simulink model "grid_afe_n"  (R2026a)
settings: Solver=ode23tb  StopTime=simlength  FixedStep=tc  MaxStep=glb_time.tc
values from neighbouring files (symbols this model uses):
  afe_ctrl = ctrl_afe_setup(glb_time.ts_afe, grid_emu.omega_grid_nom)    [init_model.m]
  afe_pwm_phase_shift_mod1 = 0    [init_model.m]
  afe_pwm_phase_shift_mod2 = 0    [init_model.m]
  afe_pwm_phase_shift_mod3 = 0    [init_model.m]
  afe_pwm_phase_shift_mod4 = 0    [init_model.m]
  filters = setup_global_filters(glb_time.ts_afe, glb_time.ts_inv, glb_time.ts_dab, glb_time.tc)    [init_model.m]
  frt_data = frt_settings(test_index, test_subindex, asymmetric_error_type,      enable_frt_1, enable_frt_2, start_time_LVRT, deepPOSxi, deepPOSeta, deepNEGxi, deepNEGeta)    [init_model.m]
  glb_time = timing_setup(fpwm_afe, trgo_afe, fpwm_inv, trgo_inv, fpwm_single_phase_inv, trgo_single_phase_inv, fpwm_dab, trgo_dab,      fpwm_psfbc, trgo_psfbc, fpwm_isop_rail, trgo_isop_rail, fpwm_cllc, trgo_cllc, t_measure, tc_factor, tc_decimation, delay_pwm, dead_time_afe,      dead_time_inv, dead_time_single_phase_inv, dead_time_dab, dead_time_psfbc, dead_time_isop_rail, dead_time_cllc)    [init_model.m]
  grid_emu = grid_three_phase_emulator('Dyn11', delta_star, grid_nominal_power, application_voltage, us1, us2, fgrid,                  eq_grid_inductance, eq_grid_resistance, eta, ucc, i1m, p_iron, n1, n2, core_area, core_length, mur,                  up_xi_pu_ref, up_eta_pu_ref, un_xi_pu_ref, un_eta_pu_ref)    [init_model.m]
  i_react_pos_ref_2 = -ixi_ref_mod1*tan(acos(0.95))    [init_model.m]
  i_react_pos_ref_3 = ixi_ref_mod1*tan(acos(0.95))    [init_model.m]
  ixi_ref_mod1 = -0.85    [init_model.m]
  ixi_ref_mod2 = -0.85    [init_model.m]
  ixi_ref_mod3 = -0.85    [init_model.m]
  ixi_ref_mod4 = -0.85    [init_model.m]
  ki_align = 18    [init_model.m]
  kp_align = 0.25    [init_model.m]
  lim_down_align = -0.05    [init_model.m]
  lim_up_align = 0.05    [init_model.m]
  mavarage_filter_frequency_base_order = 2    [init_model.m]
  time_gain_afe_module_1 = 1.0002    [init_model.m]
  time_gain_afe_module_2 = 1.0015    [init_model.m]
  time_gain_afe_module_3 = 0.9988    [init_model.m]
  time_gain_afe_module_4 = 1.0020    (= 1.002)    [init_model.m]
  time_i_react_pos_ref_1 = start_time_LVRT + error_length + 0.335    [init_model.m]
  time_i_react_pos_ref_2 = time_i_react_pos_ref_1 + 0.5    (= 0.5)    [init_model.m]
  u_cm_comp_mod1 = 0    [init_model.m]
  u_cm_comp_mod2 = -1    [init_model.m]
  u_cm_comp_mod3 = -1    [init_model.m]
  u_cm_comp_mod4 = -1    [init_model.m]
undefined symbols (not defined in the file or in its folder): hwdata, magnitude
libraries: fl_lib x113, nesl_utility x75, moving_average_filter x40, moving_average_filter_cc x32, sl_discontinuities x12, linear_double_integrator_observer_ccaller x8, discrete_time_low_pass_filter x4, threephase_inductor_lib x4, dclink_for_two_levels x4, three_phase_pwm_modulator x4, three_phase_inverter_ideal_switch_based_model x4, three_phase_inverter_igbt_advanced_thermal_model x4
(part 8 of 19)

== system grid_afe_n/afe_abc_mod2/AFE_control/afe_control/current_ctrl/inner_current_ctrl ==
  In1 : Inport
  is_abc : Inport  Port=2
  Mux : Mux  Inputs=3
  Selector : Selector  InputPortWidth=3  IndexOptions=Index vector (dialog)  Indices=[1]  OutputSizes=1
  Selector1 : Selector  InputPortWidth=3  IndexOptions=Index vector (dialog)  Indices=[1]  OutputSizes=1
  Selector2 : Selector  InputPortWidth=3  IndexOptions=Index vector (dialog)  Indices=[2]  OutputSizes=1
  Selector3 : Selector  InputPortWidth=3  IndexOptions=Index vector (dialog)  Indices=[2]  OutputSizes=1
  Selector4 : Selector  InputPortWidth=3  IndexOptions=Index vector (dialog)  Indices=[3]  OutputSizes=1
  Selector5 : Selector  InputPortWidth=3  IndexOptions=Index vector (dialog)  Indices=[3]  OutputSizes=1
  isa_ref/isa : Scope  NumInputPorts=2
      settings: ActiveDisplayYMinimum=-3.12274169921875  ActiveDisplayYMaximum=3.67108154296875
  isb_ref/isb : Scope  NumInputPorts=2
      settings: ActiveDisplayYMinimum=-2.378662109375  ActiveDisplayYMaximum=2.814208984375  DataLoggingVariableName=ScopeData2
  isc_ref/isc : Scope  NumInputPorts=2
      settings: ActiveDisplayYMinimum=-2.90966796875  ActiveDisplayYMaximum=2.88134765625  DataLoggingVariableName=ScopeData3
  rpi_phase_a : Subsystem
  rpi_phase_b : Subsystem
  rpi_phase_c : Subsystem
  zero_current_ctrl : Subsystem
  uabg : Outport  VectorParamsAs1DForOutWhenUnconnected=off
  tag scope: isa=scoped, isa_ref=scoped, isb=scoped, isb_ref=scoped, isc=scoped, isc_ref=scoped
  wires:
  zero_current_ctrl/1(u_ctrl_out) -> uabg/1
  Mux/1 -> zero_current_ctrl/1(d_abc)  "d_abc"
  rpi_phase_c/1(Out1) -> Mux/3  "dc"
  rpi_phase_b/1(Out1) -> Mux/2  "db"
  rpi_phase_a/1(Out1) -> Mux/1  "da"
  Selector5/1 -> isc_ref/isc/2, [isc], rpi_phase_c/2(In2)  "isc"
  Selector4/1 -> isc_ref/isc/1, [isc_ref], rpi_phase_c/1(In1)  "isc_ref"
  Selector3/1 -> isb_ref/isb/2, [isb], rpi_phase_b/2(In2)  "isb"
  Selector2/1 -> isb_ref/isb/1, [isb_ref], rpi_phase_b/1(In1)  "isb_ref"
  Selector1/1 -> rpi_phase_a/2(In2), isa_ref/isa/2, [isa]  "isa"
  Selector/1 -> rpi_phase_a/1(In1), isa_ref/isa/1, [isa_ref]  "isa_ref"
  is_abc/1 -> Selector1/1, Selector3/1, Selector5/1  "id_abc"
  In1/1 -> Selector/1, Selector2/1, Selector4/1  "id_abc_ref"

== system grid_afe_n/afe_abc_mod2/AFE_control/afe_control/current_ctrl/xieta2abc ==
  pos_xi : Inport
  pos_eta : Inport  Port=2
  neg_xi : Inport  Port=3
  neg_eta : Inport  Port=4
  phase : Inport  Port=5
  MATLAB Function2 : MATLAB Function  TreatAsAtomicUnit=on
  Mux : Mux  Inputs=3
  Negative Sequence : MATLAB Function  TreatAsAtomicUnit=on
  Positive Sequence : MATLAB Function  TreatAsAtomicUnit=on
  Sum : Sum  Inputs=|++
  Sum1 : Sum  Inputs=|++
  i_abc : Outport
  wires:
  Mux/1 -> i_abc/1  "i_abc"
  pos_eta/1 -> Positive Sequence/2(eta)
  pos_xi/1 -> Positive Sequence/1(xi)
  neg_xi/1 -> Negative Sequence/1(xi)
  Sum1/1 -> MATLAB Function2/2(beta)
  MATLAB Function2/2(b) -> Mux/2  "i_b"
  Negative Sequence/2(beta) -> Sum1/2
  Positive Sequence/1(alpha) -> Sum/1
  Negative Sequence/1(alpha) -> Sum/2
  MATLAB Function2/3(c) -> Mux/3  "i_c"
  phase/1 -> Positive Sequence/3(phase), Negative Sequence/3(phase)
  Sum/1 -> MATLAB Function2/1(alpha)
  Positive Sequence/2(beta) -> Sum1/1
  MATLAB Function2/1(a) -> Mux/1  "i_a"
  neg_eta/1 -> Negative Sequence/2(eta)

== system grid_afe_n/afe_abc_mod2/AFE_control/afe_control/data_to_worspace_module_1/dq_pll ==
  Bus Creator1 : BusCreator  Inputs=8
  dqPLLs : Outport
  wires:
  [phase_grid_fht_simulink_pll] -> Bus Creator1/5  "phase_grid_fht_simulink_pll"
  [omega_grid_fht_simulink_pll] -> Bus Creator1/6  "omega_grid_fht_simulink_pll"
  [omega_grid_fhtsr_dqpll] -> Bus Creator1/8  "omega_grid_fhtsr_dqpll"
  [phase_grid_fhtsr_dqpll] -> Bus Creator1/7  "phase_grid_fhtsr_dqpll"
  [omega_grid_dqpll_ccaller] -> Bus Creator1/4  "omega_grid_dqpll_ccaller"
  [phase_grid_dqpll_ccaller] -> Bus Creator1/3  "phase_grid_dqpll_ccaller"
  [omega_grid_pll_pu] -> Bus Creator1/2  "omega_grid_pu_dqpll"
  [phase_grid_pll] -> Bus Creator1/1  "phase_grid_dqpll"
  Bus Creator1/1 -> dqPLLs/1

== system grid_afe_n/afe_abc_mod2/AFE_control/afe_control/data_to_worspace_module_1/inner_current_tracking ==
  Bus Creator1 : BusCreator  Inputs=11
  m_inner_current_tracking : Outport
  wires:
  Bus Creator1/1 -> m_inner_current_tracking/1
  [isc_ref] -> Bus Creator1/7  "isc_pu_ref"
  [iz_ctrl_out] -> Bus Creator1/11  "iz_ctrl_out"
  [isb_ref] -> Bus Creator1/5  "isb_pu_ref"
  [isb] -> Bus Creator1/6  "isb_pu"
  [iz_pu_ref] -> Bus Creator1/9  "iz_pu_ref"
  [id_xi_pu] -> Bus Creator1/1  "i_xi_pu"
  [isa] -> Bus Creator1/4  "isa_pu"
  [isa_ref] -> Bus Creator1/3  "isa_pu_ref"
  [isc] -> Bus Creator1/8  "isc_pu"
  [id_eta_pu] -> Bus Creator1/2  "i_eta_pu"
  [iz_pu] -> Bus Creator1/10  "iz_pu"

== system grid_afe_n/afe_abc_mod2/AFE_control/afe_control/data_to_worspace_module_1/pwr_meter ==
  Bus Creator1 : BusCreator  Inputs=4
  m_pwr_meter : Outport
  wires:
  [i_grid_pu_rms] -> Bus Creator1/1  "i_grid_pu_rms"
  [pwr_react_grid] -> Bus Creator1/4  "pwr_react_grid"
  [pwr_act_grid] -> Bus Creator1/3  "pwr_act_grid"
  Bus Creator1/1 -> m_pwr_meter/1
  [u_grid_pu_rms] -> Bus Creator1/2  "u_grid_pu_rms"

== system grid_afe_n/afe_abc_mod2/AFE_control/afe_control/data_to_worspace_module_1/sequences_data ==
  Bus Creator1 : BusCreator  Inputs=11
  Bus Selector : BusSelector  OutputSignals=i_grid_pos_eta_ref,i_grid_neg_eta_ref,i_grid_neg_xi_ref
  m_seq : Outport
  wires:
  Bus Creator1/1 -> m_seq/1
  [i_grid_seq_ref] -> Bus Selector/1
  Bus Selector/3 -> Bus Creator1/3  "<i_grid_neg_xi_ref>"
  Bus Selector/2 -> Bus Creator1/2  "<i_grid_neg_eta_ref>"
  Bus Selector/1 -> Bus Creator1/1  "<i_grid_pos_eta_ref>"
  [v_grid_pos_xi_avg] -> Bus Creator1/4  "v_grid_pos_xi_avg"
  [v_grid_pos_eta_avg] -> Bus Creator1/5  "v_grid_pos_eta_avg"
  [v_grid_neg_xi_avg] -> Bus Creator1/6  "v_grid_neg_xi_avg"
  [v_grid_neg_eta_avg] -> Bus Creator1/7  "v_grid_neg_eta_avg"
  [i_grid_pos_xi_avg] -> Bus Creator1/8  "i_grid_pos_xi_avg"
  [i_grid_pos_eta_avg] -> Bus Creator1/9  "i_grid_pos_eta_avg"
  [i_grid_neg_xi_avg] -> Bus Creator1/10  "i_grid_neg_xi_avg"
  [i_grid_neg_eta_avg] -> Bus Creator1/11  "i_grid_neg_eta_avg"

== system grid_afe_n/afe_abc_mod2/AFE_control/afe_control/grid_current_sequences_and_reactive_pwr_ctrl/current_sequence_avg ==
  i_grid_pos_xi : Inport
  i_grid_pos_eta : Inport  Port=2
  i_grid_neg_xi : Inport  Port=3
  i_grid_neg_eta : Inport  Port=4
  Variant Source{,1..3} (4 alike) : VariantSource  VariantControls={use_moving_average_from_ccaller_mod3 == 1, use_moving_average_from_ccaller_mod3 == 0}
  average_filter : Subsystem
  average_filter_ccaller : Subsystem
  i_grid_pos_xi_avg : Outport
  i_grid_pos_eta_avg : Outport  Port=2
  i_grid_neg_xi_avg : Outport  Port=3
  i_grid_neg_eta_avg : Outport  Port=4
  wires:
  average_filter_ccaller/4(i_grid_neg_eta_avg) -> Variant Source3/1
  average_filter_ccaller/3(i_grid_neg_xi_avg) -> Variant Source2/1
  average_filter_ccaller/2(i_grid_pos_eta_avg) -> Variant Source1/1
  average_filter/4(i_grid_neg_eta_avg) -> Variant Source3/2
  average_filter/3(i_grid_neg_xi_avg) -> Variant Source2/2
  average_filter/2(i_grid_pos_eta_avg) -> Variant Source1/2
  average_filter/1(i_grid_pos_xi_avg) -> Variant Source/2
  average_filter_ccaller/1(i_grid_pos_xi_avg) -> Variant Source/1
  Variant Source1/1 -> i_grid_pos_eta_avg/1
  Variant Source2/1 -> i_grid_neg_xi_avg/1
  Variant Source3/1 -> i_grid_neg_eta_avg/1
  Variant Source/1 -> i_grid_pos_xi_avg/1
  i_grid_neg_eta/1 -> average_filter_ccaller/4(i_grid_neg_eta), average_filter/4(i_grid_neg_eta)
  i_grid_neg_xi/1 -> average_filter_ccaller/3(i_grid_neg_xi), average_filter/3(i_grid_neg_xi)
  i_grid_pos_eta/1 -> average_filter_ccaller/2(i_grid_pos_eta), average_filter/2(i_grid_pos_eta)
  i_grid_pos_xi/1 -> average_filter_ccaller/1(i_grid_pos_xi), average_filter/1(i_grid_pos_xi)

== system grid_afe_n/afe_abc_mod2/AFE_control/afe_control/grid_current_sequences_and_reactive_pwr_ctrl/grid_current_sampling_and_alpha_beta_transformation ==
  ig_abc : Inport
  i_abc2alphabeta : MATLAB Function  TreatAsAtomicUnit=on
  i_grid_alpha : Outport
  i_grid_beta : Outport  Port=2
  wires:
  ig_abc/1 -> i_abc2alphabeta/1(i_abc)
  i_abc2alphabeta/1(alpha) -> i_grid_alpha/1  "i_grid_alpha"
  i_abc2alphabeta/2(beta) -> i_grid_beta/1  "i_grid_beta"

== system grid_afe_n/afe_abc_mod2/AFE_control/afe_control/grid_current_sequences_and_reactive_pwr_ctrl/i_alphabeta2xieta ==
  alpha : Inport
  beta : Inport  Port=2
  gamma : Inport  Port=3
  MATLAB Function : MATLAB Function  TreatAsAtomicUnit=on
  MATLAB Function1 : MATLAB Function  TreatAsAtomicUnit=on
  xi : Outport
  v_grid_pos_eta : Outport  Port=2
  v_grid_neg_xi : Outport  Port=3
  e : Outport  Port=4
  wires:
  MATLAB Function/1(xi) -> xi/1  "i_grid_pos_xi"
  MATLAB Function1/2(eta) -> e/1  "i_grid_neg_eta"
  MATLAB Function1/1(xi) -> v_grid_neg_xi/1  "i_grid_neg_xi"
  MATLAB Function/2(eta) -> v_grid_pos_eta/1  "i_grid_pos_eta"
  gamma/1 -> MATLAB Function/3(gamma), MATLAB Function1/3(gamma)  "gamma_grid"
  beta/1 -> MATLAB Function/2(beta), MATLAB Function1/2(beta)  "i_grid_beta"
  alpha/1 -> MATLAB Function/1(alpha), MATLAB Function1/1(alpha)  "i_grid_alpha"

== system grid_afe_n/afe_abc_mod2/AFE_control/afe_control/grid_current_sequences_and_reactive_pwr_ctrl/sequences_current_control ==
  i_pos_xi : Inport
  i_pos_eta : Inport  Port=2
  i_neg_xi : Inport  Port=3
  i_neg_eta : Inport  Port=4
  Bus Selector : BusSelector  OutputSignals=i_grid_pos_eta_ref,i_grid_neg_eta_ref,i_grid_neg_xi_ref
  Constant : Constant  Value=0
  Constant1 : Constant  Value=0
  Constant2 : Constant  Value=0
  Gain : Gain  Gain=-1
  Gain1 : Gain  Gain=-1
  Gain2 : Gain  Gain=-1
  Negative-Seq. eta-Control : Subsystem
  Negative-Seq. xi-Control : Subsystem
  Positive-Seq. eta-Control : Subsystem
  Sum : Sum  Inputs=|+-
  Sum1 : Sum  Inputs=|+-
  Sum2 : Sum  Inputs=|+-
  Terminator : Terminator
  i_neg_eta_ref/i_neg_eta : Scope  NumInputPorts=2
      settings: ActiveDisplayYMinimum=-1  ActiveDisplayYMaximum=1  DataLoggingVariableName=ScopeData6
  i_neg_xi_ref/i_neg_xi : Scope  NumInputPorts=2
      settings: ActiveDisplayYMinimum=-2.0072433506888805  ActiveDisplayYMaximum=0.71326150187789183  DataLoggingVariableName=ScopeData7
  i_pos_eta_ref/i_pos_eta : Scope  NumInputPorts=2
      settings: ActiveDisplayYMinimum=-2.9962328913117955  ActiveDisplayYMaximum=0.9969886390149818  DataLoggingVariableName=ScopeData5
  tag scope: i_stack_neg_eta_ref=scoped, i_stack_neg_xi_ref=scoped, i_stack_pos_eta_ref=scoped
  wires:
  Negative-Seq. xi-Control/1(u) -> [i_stack_neg_xi_ref]
  Negative-Seq. eta-Control/1(u) -> [i_stack_neg_eta_ref]
  Positive-Seq. eta-Control/1(u) -> [i_stack_pos_eta_ref]
  Gain2/1 -> Negative-Seq. xi-Control/2(e)
  Gain1/1 -> Negative-Seq. eta-Control/2(e)
  Gain/1 -> Positive-Seq. eta-Control/2(e)
  i_neg_xi/1 -> Sum2/2, i_neg_xi_ref/i_neg_xi/2  "i_neg_xi"
  i_neg_eta/1 -> i_neg_eta_ref/i_neg_eta/2, Sum1/2  "i_neg_eta"
  i_pos_eta/1 -> Sum/2, i_pos_eta_ref/i_pos_eta/2  "i_pos_eta"
  Sum/1 -> Gain/1
  Sum1/1 -> Gain1/1
  Sum2/1 -> Gain2/1
  Bus Selector/3 -> Sum2/1, i_neg_xi_ref/i_neg_xi/1  "<i_grid_neg_xi_ref>"
  Bus Selector/2 -> Sum1/1, i_neg_eta_ref/i_neg_eta/1  "<i_grid_neg_eta_ref>"
  Bus Selector/1 -> Sum/1, i_pos_eta_ref/i_pos_eta/1  "<i_grid_pos_eta_ref>"
  [i_grid_seq_ref] -> Bus Selector/1
  i_pos_xi/1 -> Terminator/1
  Constant/1 -> Positive-Seq. eta-Control/1(ff)
  Constant1/1 -> Negative-Seq. eta-Control/1(ff)
  Constant2/1 -> Negative-Seq. xi-Control/1(ff)

== system grid_afe_n/afe_abc_mod2/AFE_control/afe_control/grid_voltage_phase_lock_loops/FHT-PLL ==
  ug_abc_pu : Inport
  pll_stageA : Subsystem
  pll_stageB : Subsystem
  gamma_grid_fht_pll : Outport
  omega_grid_fht_pll : Outport  Port=2
  wires:
  pll_stageB/1(gamma_grid_ddsrf_pll) -> pll_stageA/1(gamma_grid), gamma_grid_fht_pll/1
  pll_stageA/2(u_grid_eta) -> pll_stageB/2(u_grid_pos_eta)  "u_grid_pos_eta"
  pll_stageA/1(u_grid_xi) -> pll_stageB/1(u_grid_pos_xi)  "u_grid_pos_xi"
  pll_stageB/2(omega_grid_ddsrf_pll) -> omega_grid_fht_pll/1
  ug_abc_pu/1 -> pll_stageA/2(ug_abc_pu)

== system grid_afe_n/afe_abc_mod2/AFE_control/afe_control/grid_voltage_phase_lock_loops/FHT-PLL_simulink ==
  ug_abc_pu : Inport
  Goto Tag Visibility55 : GotoTagVisibility  GotoTag=Vgrid_unorm_fht_simulink
  pll_stageA : Subsystem
  pll_stageB : Subsystem
  gamma_grid_fht_pll : Outport
  omega_grid_fht_pll : Outport  Port=2
  wires:
  pll_stageB/1(gamma_grid_ddsrf_pll) -> pll_stageA/1(gamma_grid), gamma_grid_fht_pll/1
  pll_stageA/2(u_grid_eta) -> pll_stageB/2(u_grid_pos_eta)  "u_grid_pos_eta"
  pll_stageA/1(u_grid_xi) -> pll_stageB/1(u_grid_pos_xi)  "u_grid_pos_xi"
  pll_stageB/2(omega_grid_ddsrf_pll) -> omega_grid_fht_pll/1
  ug_abc_pu/1 -> pll_stageA/2(ug_abc_pu)

== system grid_afe_n/afe_abc_mod2/AFE_control/afe_control/grid_voltage_phase_lock_loops/dq_pll ==
  ug_abc_pu : Inport
  Goto Tag Visibility1 : GotoTagVisibility  GotoTag=Vgrid_unorm_dqpll
  pll_stageA : Subsystem
  pll_stageB : Subsystem
  phase_grid_dqpll : Outport
  omega_grid_pu_dqpll : Outport  Port=2
  wires:
  ug_abc_pu/1 -> pll_stageA/2(ug_abc)
  pll_stageB/2(omega_grid_pu_pll) -> omega_grid_pu_dqpll/1
  pll_stageA/1(u_grid_pos_xi) -> pll_stageB/1(u_grid_pos_xi)  "u_grid_pos_xi"
  pll_stageB/1(phase_grid_pll) -> pll_stageA/1(phase_grid), phase_grid_dqpll/1
  pll_stageA/2(u_grid_pos_eta) -> pll_stageB/2(u_grid_pos_eta)  "u_grid_pos_eta"

== system grid_afe_n/afe_abc_mod2/AFE_control/afe_control/grid_voltage_phase_lock_loops/dq_pll_ccaller ==
  ug_abc_pu : Inport
  Bus Selector : BusSelector  OutputSignals=omega_pu_hat,gamma_hat,u_grid_xi,u_grid_eta,dqpll_pll_state
  C Caller : CCaller  FunctionName=dqpll_grid_process_simulink  PortSpecificationStruct="%)30     .    N H   8    (     @         %    \"     8    !     0         %  0 \"0    $    _    07)G3F%M90  4&]R=$YA;64 4V-O<&4     26YD97@     5'EP90      4VEZ90      27-';&]B86P   X    P    !@    @    $          4    (     0    ,    !         !   P!O=70 #@   #     &    \"     0         !0    @    !     P    $         $  # &]U=  .    .     8    (    !          %    \"     $    &     0         0   ...(+3319 chars)"
  Constant : Constant  Value=glb_time.ts_afe
  Data Type Conversion{1..2,4..5} (4 alike) : DataTypeConversion  OutDataTypeStr=single  SaturateOnIntegerOverflow=off  RndMeth=Floor
  Data Type Conversion{6..10} (5 alike) : DataTypeConversion  OutDataTypeStr=double  SaturateOnIntegerOverflow=off  RndMeth=Floor
  Data Type Conversion3 : DataTypeConversion  OutDataTypeStr=uint8  SaturateOnIntegerOverflow=off  RndMeth=Floor
  Demux : Demux  Outputs=3
  Step : Step  Time=0.01  InitialValue=1  FinalValue=0
  first_harmonic_tracker : Scope  NumInputPorts=3
      settings: ActiveDisplayYMinimum=-1.7184470891952515  ActiveDisplayYMaximum=1.8384636640548706
  first_harmonic_tracker_phase_u : Subsystem
  first_harmonic_tracker_phase_v : Subsystem
  first_harmonic_tracker_phase_w : Subsystem
  gamma_hat : Outport  VectorParamsAs1DForOutWhenUnconnected=off
  omega_pu_hat : Outport  Port=2  VectorParamsAs1DForOutWhenUnconnected=off
  dqpll_uxi : Outport  Port=3  VectorParamsAs1DForOutWhenUnconnected=off
  dqpll_ueta : Outport  Port=4  VectorParamsAs1DForOutWhenUnconnected=off
  dqpll_state : Outport  Port=5  VectorParamsAs1DForOutWhenUnconnected=off
  wires:
  first_harmonic_tracker_phase_w/1(u_hat) -> Data Type Conversion5/1, first_harmonic_tracker/3  "tracker_phase_w"
  first_harmonic_tracker_phase_v/1(u_hat) -> Data Type Conversion4/1, first_harmonic_tracker/2  "tracker_phase_v"
  first_harmonic_tracker_phase_u/1(u_hat) -> Data Type Conversion2/1, first_harmonic_tracker/1  "tracker_phase_u"
  Data Type Conversion6/1 -> omega_pu_hat/1
  Demux/3 -> first_harmonic_tracker_phase_w/1(u)
  Demux/2 -> first_harmonic_tracker_phase_v/1(u)
  Demux/1 -> first_harmonic_tracker_phase_u/1(u)
  ug_abc_pu/1 -> Demux/1
  Data Type Conversion9/1 -> dqpll_ueta/1
  Data Type Conversion8/1 -> dqpll_uxi/1
  Data Type Conversion10/1 -> dqpll_state/1
  Data Type Conversion7/1 -> gamma_hat/1
  Bus Selector/5 -> Data Type Conversion10/1  "<dqpll_pll_state>"
  Bus Selector/4 -> Data Type Conversion9/1  "<u_grid_eta>"
  Bus Selector/3 -> Data Type Conversion8/1  "<u_grid_xi>"
  Bus Selector/2 -> Data Type Conversion7/1  "<gamma_hat>"
  Bus Selector/1 -> Data Type Conversion6/1  "<omega_pu_hat>"
  C Caller/1 -> Bus Selector/1
  Data Type Conversion1/1 -> C Caller/5
  Data Type Conversion5/1 -> C Caller/4
  Data Type Conversion4/1 -> C Caller/3
  Data Type Conversion2/1 -> C Caller/2
  Data Type Conversion3/1 -> C Caller/1
  Constant/1 -> Data Type Conversion1/1
  Step/1 -> Data Type Conversion3/1

== system grid_afe_n/afe_abc_mod2/AFE_control/afe_control/grid_voltage_sequences/grid_voltage_sampling_and_alpha_beta_transformation ==
  v_abc : Inport
  v_abc2alphabeta : MATLAB Function  TreatAsAtomicUnit=on
  u_grid_alpha : Outport
  u_grid_beta : Outport  Port=2
  wires:
  v_abc/1 -> v_abc2alphabeta/1(v_abc)
  v_abc2alphabeta/2(beta) -> u_grid_beta/1  "u_grid_beta"
  v_abc2alphabeta/1(alpha) -> u_grid_alpha/1  "u_grid_alpha"

== system grid_afe_n/afe_abc_mod2/AFE_control/afe_control/grid_voltage_sequences/v_alphabeta2xieta ==
  alpha : Inport
  beta : Inport  Port=2
  gamma : Inport  Port=3
  MATLAB Function : MATLAB Function  TreatAsAtomicUnit=on
  MATLAB Function1 : MATLAB Function  TreatAsAtomicUnit=on
  xi : Outport
  eta : Outport  Port=2
  v_grid_neg_xi : Outport  Port=3
  v_grid_neg_eta : Outport  Port=4
  wires:
  MATLAB Function1/2(eta) -> v_grid_neg_eta/1  "u_grid_neg_eta"
  MATLAB Function1/1(xi) -> v_grid_neg_xi/1  "u_grid_neg_xi"
  MATLAB Function/2(eta) -> eta/1  "u_grid_pos_eta"
  MATLAB Function/1(xi) -> xi/1  "u_grid_pos_xi"
  gamma/1 -> MATLAB Function/3(gamma), MATLAB Function1/3(gamma)  "gamma_grid"
  beta/1 -> MATLAB Function/2(beta), MATLAB Function1/2(beta)  "u_grid_beta"
  alpha/1 -> MATLAB Function/1(alpha), MATLAB Function1/1(alpha)  "u_grid_alpha"

== system grid_afe_n/afe_abc_mod2/AFE_control/afe_control/grid_voltage_sequences/voltage_sequence_avg ==
  v_grid_pos_xi : Inport
  v_grid_pos_eta : Inport  Port=2
  v_grid_neg_xi : Inport  Port=3
  v_grid_neg_eta : Inport  Port=4
  Variant Source{1..4} (4 alike) : VariantSource  VariantControls={use_moving_average_from_ccaller_mod2 == 1, use_moving_average_from_ccaller_mod2 == 0}
  average_filter : Subsystem
  average_filter_ccaller : Subsystem
  v_grid_pos_xi_avg : Outport
  v_grid_pos_eta_avg : Outport  Port=2
  v_grid_neg_xi_avg : Outport  Port=3
  v_grid_neg_eta_avg : Outport  Port=4
  wires:
  average_filter/4(v_grid_neg_eta_avg) -> Variant Source3/2
  average_filter/3(v_grid_neg_xi_avg) -> Variant Source2/2
  average_filter/2(v_grid_pos_eta_avg) -> Variant Source1/2
  average_filter/1(v_grid_pos_xi_avg) -> Variant Source4/2
  average_filter_ccaller/4(v_grid_neg_eta_avg) -> Variant Source3/1
  average_filter_ccaller/3(v_grid_neg_xi_avg) -> Variant Source2/1
  average_filter_ccaller/2(v_grid_pos_eta_avg) -> Variant Source1/1
  average_filter_ccaller/1(v_grid_pos_xi_avg) -> Variant Source4/1
  Variant Source3/1 -> v_grid_neg_eta_avg/1
  Variant Source2/1 -> v_grid_neg_xi_avg/1
  Variant Source1/1 -> v_grid_pos_eta_avg/1
  Variant Source4/1 -> v_grid_pos_xi_avg/1
  v_grid_neg_eta/1 -> average_filter/4(v_grid_neg_eta), average_filter_ccaller/4(v_grid_neg_eta)
  v_grid_neg_xi/1 -> average_filter/3(v_grid_neg_xi), average_filter_ccaller/3(v_grid_neg_xi)
  v_grid_pos_eta/1 -> average_filter/2(v_grid_pos_eta), average_filter_ccaller/2(v_grid_pos_eta)
  v_grid_pos_xi/1 -> average_filter_ccaller/1(v_grid_pos_xi), average_filter/1(v_grid_pos_xi)

== system grid_afe_n/afe_abc_mod2/AFE_control/afe_control/ig afe quantizzation and one step delay/ig afe quantizzation and one step delay ==
  ig_u_pu : Inport
  ig_v_pu : Inport  Port=2
  ig_w_pu : Inport  Port=3
  Gain4 : Gain  Gain=-1
  Gain5 : Gain  Gain=-1
  Gain6 : Gain  Gain=-1
  Quantizer1 : Quantizer  QuantizationInterval=adc_quantization
  Quantizer2 : Quantizer  QuantizationInterval=adc_quantization
  Quantizer4 : Quantizer  QuantizationInterval=adc_quantization
  Unit Delay : UnitDelay  SampleTime=-1
  Unit Delay1 : UnitDelay  SampleTime=-1
  Unit Delay2 : UnitDelay  SampleTime=-1
  Zero-Order Hold : ZeroOrderHold  SampleTime=-1
  Zero-Order Hold1 : ZeroOrderHold  SampleTime=-1
  Zero-Order Hold2 : ZeroOrderHold  SampleTime=-1
  igd_u_pu : Outport
  igd_v_pu : Outport  Port=2
  igd_w_pu : Outport  Port=3
  wires:
  Zero-Order Hold2/1 -> Quantizer2/1
  Zero-Order Hold1/1 -> Quantizer1/1
  Zero-Order Hold/1 -> Quantizer4/1
  Gain6/1 -> igd_w_pu/1
  Gain5/1 -> igd_v_pu/1
  Gain4/1 -> igd_u_pu/1
  Unit Delay2/1 -> Gain6/1
  Unit Delay1/1 -> Gain5/1
  Unit Delay/1 -> Gain4/1
  ig_w_pu/1 -> Zero-Order Hold2/1
  ig_v_pu/1 -> Zero-Order Hold1/1
  ig_u_pu/1 -> Zero-Order Hold/1
  Quantizer2/1 -> Unit Delay2/1
  Quantizer4/1 -> Unit Delay/1
  Quantizer1/1 -> Unit Delay1/1

== system grid_afe_n/afe_abc_mod2/AFE_control/afe_control/instantaneus_power/abc2alphabeta ==
  a : Inport
  b : Inport  Port=2
  c : Inport  Port=3
  Gain1 : Gain  Gain=-1/2
  Gain11 : Gain  Gain=-1/2
  Gain2 : Gain  Gain=0
  Gain3 : Gain  Gain=sqrt(3)/2
  Gain4 : Gain  Gain=-sqrt(3)/2
  Gain8 : Gain  Gain=2/3
  Gain9 : Gain  Gain=2/3
  Sum : Sum  Inputs=+++
  Sum1 : Sum  Inputs=+++
  "alpha " : Outport  VectorParamsAs1DForOutWhenUnconnected=off
  "beta " : Outport  Port=2  VectorParamsAs1DForOutWhenUnconnected=off
  wires:
  a/1 -> Sum/1, Gain2/1
  Gain1/1 -> Sum/3
  b/1 -> Gain11/1, Gain3/1
  Gain9/1 -> "beta "/1
  c/1 -> Gain1/1, Gain4/1
  Sum/1 -> Gain8/1
  Gain8/1 -> "alpha "/1
  Sum1/1 -> Gain9/1
  Gain4/1 -> Sum1/3
  Gain11/1 -> Sum/2
  Gain2/1 -> Sum1/1
  Gain3/1 -> Sum1/2

== system grid_afe_n/afe_abc_mod2/AFE_control/afe_control/instantaneus_power/abc2alphabeta  ==
  a : Inport
  b : Inport  Port=2
  c : Inport  Port=3
  Gain1 : Gain  Gain=-1/2
  Gain11 : Gain  Gain=-1/2
  Gain2 : Gain  Gain=0
  Gain3 : Gain  Gain=sqrt(3)/2
  Gain4 : Gain  Gain=-sqrt(3)/2
  Gain8 : Gain  Gain=2/3
  Gain9 : Gain  Gain=2/3
  Sum : Sum  Inputs=+++
  Sum1 : Sum  Inputs=+++
  "alpha " : Outport  VectorParamsAs1DForOutWhenUnconnected=off
  "beta " : Outport  Port=2  VectorParamsAs1DForOutWhenUnconnected=off
  wires:
  b/1 -> Gain3/1, Gain11/1
  Gain8/1 -> "alpha "/1
  Gain4/1 -> Sum1/3
  Gain3/1 -> Sum1/2
  Gain1/1 -> Sum/3
  Sum1/1 -> Gain9/1
  Sum/1 -> Gain8/1
  c/1 -> Gain4/1, Gain1/1
  Gain11/1 -> Sum/2
  Gain9/1 -> "beta "/1
  Gain2/1 -> Sum1/1
  a/1 -> Gain2/1, Sum/1

== system grid_afe_n/afe_abc_mod2/AFE_control/afe_control/instantaneus_power/moving_avarage_p ==
  in : Inport
  Gain : Gain  Gain=afe_ctrl.rms.n1-1
  Gain1 : Gain  Gain=1/afe_ctrl.rms.n1
  Sum : Sum  Inputs=|++
  Unit Delay : UnitDelay  SampleTime=-1
  out : Outport  VectorParamsAs1DForOutWhenUnconnected=off
  wires:
  Sum/1 -> Gain1/1
  Unit Delay/1 -> Gain/1
  in/1 -> Sum/1
  Gain1/1 -> Unit Delay/1, out/1
  Gain/1 -> Sum/2

== system grid_afe_n/afe_abc_mod2/AFE_control/afe_control/instantaneus_power/moving_avarage_q ==
  in : Inport
  Gain : Gain  Gain=afe_ctrl.rms.n1-1
  Gain1 : Gain  Gain=1/afe_ctrl.rms.n1
  Sum : Sum  Inputs=|++
  Unit Delay : UnitDelay  SampleTime=-1
  out : Outport  VectorParamsAs1DForOutWhenUnconnected=off
  wires:
  Gain/1 -> Sum/2
  Gain1/1 -> out/1, Unit Delay/1
  in/1 -> Sum/1
  Unit Delay/1 -> Gain/1
  Sum/1 -> Gain1/1

== system grid_afe_n/afe_abc_mod2/AFE_control/afe_control/instantaneus_power/rms ==
  In1 : Inport
  Gain : Gain  Gain=afe_ctrl.rms.n10-1
  Gain1 : Gain  Gain=1/afe_ctrl.rms.n10
  Math Function : Math  Operator=magnitude^2  SignedPower=on
  Sqrt : Sqrt
  Sum : Sum  Inputs=|++
  Unit Delay : UnitDelay  SampleTime=-1
  Out1 : Outport  VectorParamsAs1DForOutWhenUnconnected=off
  wires:
  Gain/1 -> Sum/2
  Sqrt/1 -> Out1/1
  Math Function/1 -> Sum/1
  Unit Delay/1 -> Gain/1
  Gain1/1 -> Unit Delay/1, Sqrt/1
  Sum/1 -> Gain1/1
  In1/1 -> Math Function/1

== system grid_afe_n/afe_abc_mod2/AFE_control/afe_control/instantaneus_power/rms1 ==
  In1 : Inport
  Gain : Gain  Gain=afe_ctrl.rms.n10-1
  Gain1 : Gain  Gain=1/afe_ctrl.rms.n10
  Math Function : Math  Operator=magnitude^2  SignedPower=on
  Sqrt : Sqrt
  Sum : Sum  Inputs=|++
  Unit Delay : UnitDelay  SampleTime=-1
  Out1 : Outport  VectorParamsAs1DForOutWhenUnconnected=off
  wires:
  In1/1 -> Math Function/1
  Sum/1 -> Gain1/1
  Gain1/1 -> Sqrt/1, Unit Delay/1
  Unit Delay/1 -> Gain/1
  Math Function/1 -> Sum/1
  Sqrt/1 -> Out1/1
  Gain/1 -> Sum/2

== system grid_afe_n/afe_abc_mod2/AFE_control/afe_control/instantaneus_power/rms2 ==
  In1 : Inport
  Gain : Gain  Gain=afe_ctrl.rms.n10-1
  Gain1 : Gain  Gain=1/afe_ctrl.rms.n10
  Math Function : Math  Operator=magnitude^2  SignedPower=on
  Sqrt : Sqrt
  Sum : Sum  Inputs=|++
  Unit Delay : UnitDelay  SampleTime=-1
  Out1 : Outport  VectorParamsAs1DForOutWhenUnconnected=off
  wires:
  Gain/1 -> Sum/2
  Sqrt/1 -> Out1/1
  Math Function/1 -> Sum/1
  Unit Delay/1 -> Gain/1
  Gain1/1 -> Unit Delay/1, Sqrt/1
  Sum/1 -> Gain1/1
  In1/1 -> Math Function/1

== system grid_afe_n/afe_abc_mod2/AFE_control/afe_control/instantaneus_power/rms3 ==
  In1 : Inport
  Gain : Gain  Gain=afe_ctrl.rms.n10-1
  Gain1 : Gain  Gain=1/afe_ctrl.rms.n10
  Math Function : Math  Operator=magnitude^2  SignedPower=on
  Sqrt : Sqrt
  Sum : Sum  Inputs=|++
  Unit Delay : UnitDelay  SampleTime=-1
  Out1 : Outport  VectorParamsAs1DForOutWhenUnconnected=off
  wires:
  In1/1 -> Math Function/1
  Sum/1 -> Gain1/1
  Gain1/1 -> Sqrt/1, Unit Delay/1
  Unit Delay/1 -> Gain/1
  Math Function/1 -> Sum/1
  Sqrt/1 -> Out1/1
  Gain/1 -> Sum/2

== system grid_afe_n/afe_abc_mod2/AFE_control/afe_control/instantaneus_power/rms4 ==
  In1 : Inport
  Gain : Gain  Gain=afe_ctrl.rms.n10-1
  Gain1 : Gain  Gain=1/afe_ctrl.rms.n10
  Math Function : Math  Operator=magnitude^2  SignedPower=on
  Sqrt : Sqrt
  Sum : Sum  Inputs=|++
  Unit Delay : UnitDelay  SampleTime=-1
  Out1 : Outport  VectorParamsAs1DForOutWhenUnconnected=off
  wires:
  Gain/1 -> Sum/2
  Sqrt/1 -> Out1/1
  Math Function/1 -> Sum/1
  Unit Delay/1 -> Gain/1
  Gain1/1 -> Unit Delay/1, Sqrt/1
  Sum/1 -> Gain1/1
  In1/1 -> Math Function/1

== system grid_afe_n/afe_abc_mod2/AFE_control/afe_control/instantaneus_power/rms5 ==
  In1 : Inport
  Gain : Gain  Gain=afe_ctrl.rms.n10-1
  Gain1 : Gain  Gain=1/afe_ctrl.rms.n10
  Math Function : Math  Operator=magnitude^2  SignedPower=on
  Sqrt : Sqrt
  Sum : Sum  Inputs=|++
  Unit Delay : UnitDelay  SampleTime=-1
  Out1 : Outport  VectorParamsAs1DForOutWhenUnconnected=off
  wires:
  In1/1 -> Math Function/1
  Sum/1 -> Gain1/1
  Gain1/1 -> Sqrt/1, Unit Delay/1
  Unit Delay/1 -> Gain/1
  Math Function/1 -> Sum/1
  Sqrt/1 -> Out1/1
  Gain/1 -> Sum/2

== system grid_afe_n/afe_abc_mod2/AFE_control/afe_control/is afe quantizzation and one step delay/is afe quantizzation and one step delay ==
  is_u_pu : Inport
  is_v_pu : Inport  Port=2
  is_w_pu : Inport  Port=3
  Quantizer : Quantizer  QuantizationInterval=adc_quantization
  Quantizer1 : Quantizer  QuantizationInterval=adc_quantization
  Quantizer2 : Quantizer  QuantizationInterval=adc_quantization
  Unit Delay : UnitDelay  SampleTime=-1
  Unit Delay1 : UnitDelay  SampleTime=-1
  Unit Delay2 : UnitDelay  SampleTime=-1
  Zero-Order Hold : ZeroOrderHold  SampleTime=-1
  Zero-Order Hold1 : ZeroOrderHold  SampleTime=-1
  Zero-Order Hold2 : ZeroOrderHold  SampleTime=-1
  isd_u_pu : Outport
  isd_v_pu : Outport  Port=2
  isd_w_pu : Outport  Port=3
  wires:
  Zero-Order Hold2/1 -> Quantizer2/1
  Zero-Order Hold1/1 -> Quantizer1/1
  Zero-Order Hold/1 -> Quantizer/1
  is_w_pu/1 -> Zero-Order Hold2/1
  is_v_pu/1 -> Zero-Order Hold1/1
  is_u_pu/1 -> Zero-Order Hold/1
  Quantizer2/1 -> Unit Delay2/1
  Quantizer1/1 -> Unit Delay1/1
  Quantizer/1 -> Unit Delay/1
  Unit Delay2/1 -> isd_w_pu/1
  Unit Delay1/1 -> isd_v_pu/1
  Unit Delay/1 -> isd_u_pu/1

== system grid_afe_n/afe_abc_mod2/AFE_control/afe_control/islanding_mode_detector/moving_avarage_1 ==
  u : Inport
  Abs : Abs  SaturateOnIntegerOverflow=off
  Gain : Gain  Gain=afe_ctrl.omega_base * 2
  Saturation : Saturate  UpperLimit=2  LowerLimit=0.1
  dmavg_flt : moving_average_filter/dmavg_flt  ts=glb_time.ts_afe  enable_time=dmavg_filter_enable_time
  y : Outport
  wires:
  dmavg_flt/1 -> y/1
  Gain/1 -> dmavg_flt/2
  u/1 -> dmavg_flt/1
  [omega_grid_pll_pu] -> Abs/1
  Abs/1 -> Saturation/1
  Saturation/1 -> Gain/1

== system grid_afe_n/afe_abc_mod2/AFE_control/afe_control/islanding_mode_detector/moving_avarage_2 ==
  u : Inport
  Abs : Abs  SaturateOnIntegerOverflow=off
  Gain : Gain  Gain=afe_ctrl.omega_base * 2
  Saturation : Saturate  UpperLimit=2  LowerLimit=0.1
  dmavg_flt : moving_average_filter/dmavg_flt  ts=glb_time.ts_afe  enable_time=dmavg_filter_enable_time
  y : Outport
  wires:
  Saturation/1 -> Gain/1
  Abs/1 -> Saturation/1
  [omega_grid_pll_pu] -> Abs/1
  u/1 -> dmavg_flt/1
  Gain/1 -> dmavg_flt/2
  dmavg_flt/1 -> y/1

== system grid_afe_n/afe_abc_mod2/AFE_control/afe_control/phase_compensation_1/alignment_eval_afe1 ==
  local_time : Inport
  master_time : Inport  Port=2
  Constant : Constant  Value=0
  Gain : Gain  Gain=-1
  Sum : Sum  Inputs=|+-
  pi : Subsystem  mask{kp=kp_align, ki=ki_align*glb_time.ts_afe, lim_up=lim_up_align, lim_down=lim_down_align}
      mask prompts: ki "ki*ts"
      mask Display:
      | disp('pi()');
      | port_label('input', 1, 'u_ref');
      | port_label('input', 2, 'u');
      | port_label('output', 1, 'y');
  dp : Outport
  wires:
  pi/1(y) -> dp/1
  Gain/1 -> pi/2(u)
  local_time/1 -> Sum/2
  Constant/1 -> pi/1(u_ref)
  Sum/1 -> Gain/1
  master_time/1 -> Sum/1

== system grid_afe_n/afe_abc_mod2/AFE_control/afe_control/ug afe quantizzation and one step delay/ug afe quantizzation and one step delay ==
  ug_u_pu : Inport
  ug_v_pu : Inport  Port=2
  ug_w_pu : Inport  Port=3
  Quantizer1 : Quantizer  QuantizationInterval=adc_quantization
  Quantizer2 : Quantizer  QuantizationInterval=adc_quantization
  Quantizer4 : Quantizer  QuantizationInterval=adc_quantization
  Unit Delay : UnitDelay  SampleTime=-1
  Unit Delay1 : UnitDelay  SampleTime=-1
  Unit Delay2 : UnitDelay  SampleTime=-1
  Zero-Order Hold : ZeroOrderHold  SampleTime=-1
  Zero-Order Hold1 : ZeroOrderHold  SampleTime=-1
  Zero-Order Hold2 : ZeroOrderHold  SampleTime=-1
  ugd_u_pu : Outport
  ugd_v_pu : Outport  Port=2
  ugd_w_pu : Outport  Port=3
  wires:
  Zero-Order Hold2/1 -> Quantizer2/1
  Zero-Order Hold1/1 -> Quantizer1/1
  Zero-Order Hold/1 -> Quantizer4/1
  ug_u_pu/1 -> Zero-Order Hold/1
  ug_v_pu/1 -> Zero-Order Hold1/1
  ug_w_pu/1 -> Zero-Order Hold2/1
  Quantizer2/1 -> Unit Delay2/1
  Quantizer1/1 -> Unit Delay1/1
  Quantizer4/1 -> Unit Delay/1
  Unit Delay2/1 -> ugd_w_pu/1
  Unit Delay1/1 -> ugd_v_pu/1
  Unit Delay/1 -> ugd_u_pu/1

== system grid_afe_n/afe_abc_mod3/AFE_control/afe_control/FRT-VDE4110/FRT-Detection ==
  red_dyn_enabled : Inport
  LVRT_detector : MATLAB Function  TreatAsAtomicUnit=on
  Step1 : Step  Time=0.025  InitialValue=1  FinalValue=0
  Step3 : Step  Time=frt_data.settle_time  FinalValue=frt_data.enable_frt_1 + frt_data.enable_frt_2
  frt_detection_inputs mod1 : Scope  NumInputPorts=6
      settings: ActiveDisplayYMinimum=-1.0098197758197784  ActiveDisplayYMaximum=1.25924351811409  DataLoggingVariableName=ScopeData2
  voltage_rate_measure_neg : Subsystem
  voltage_rate_measure_pos : Subsystem
  frt_exceeded : Outport
  frt_state : Outport  Port=2
  red_dyn_active : Outport  Port=3
  frt_active : Outport  Port=4
  pwr_lim_enable : Outport  Port=5
  wires:
  [v_grid_neg_xi_avg] -> frt_detection_inputs mod1/2, LVRT_detector/2(vxi_n), voltage_rate_measure_neg/1(v_grid_neg_xi_avg)  "v_grid_neg_xi_avg"
  [v_grid_pos_xi_avg] -> voltage_rate_measure_pos/1(v_grid_pos_xi_avg), LVRT_detector/1(vxi_p), frt_detection_inputs mod1/1  "v_grid_pos_xi_avg"
  [v_grid_neg_eta_avg] -> frt_detection_inputs mod1/3, LVRT_detector/3(veta_n)  "v_grid_neg_eta_avg"
  Step3/1 -> frt_detection_inputs mod1/6, LVRT_detector/6(enable)  "enable"
  LVRT_detector/1(pwr_lim_enable) -> pwr_lim_enable/1  "pwr_lim_enable"
  Step1/1 -> LVRT_detector/8(reset)
  red_dyn_enabled/1 -> LVRT_detector/7(red_dyn_enabled)
  LVRT_detector/2(frt_exceeded) -> frt_exceeded/1  "lvrt_exceeded"
  LVRT_detector/5(red_dyn_active) -> red_dyn_active/1
  LVRT_detector/4(frt_state) -> frt_state/1
  LVRT_detector/3(frt_active) -> frt_active/1
  voltage_rate_measure_pos/1(vxi_pos_dot) -> frt_detection_inputs mod1/4, LVRT_detector/4(vxi_p_dot)
  voltage_rate_measure_neg/1(vxi_neg_dot) -> frt_detection_inputs mod1/5, LVRT_detector/5(vxi_n_dot)

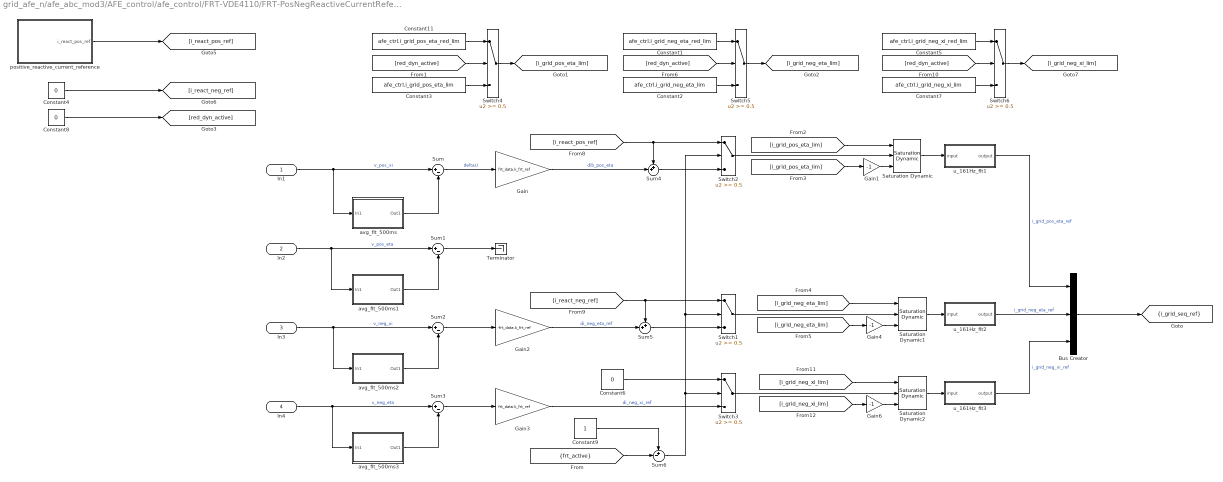
== system grid_afe_n/afe_abc_mod3/AFE_control/afe_control/FRT-VDE4110/FRT-PosNegReactiveCurrentReferences ==
  In1 : Inport
  In2 : Inport  Port=2
  In3 : Inport  Port=3
  In4 : Inport  Port=4
  Bus Creator : BusCreator  Inputs=3
  Constant1 : Constant  Value=afe_ctrl.i_grid_neg_eta_red_lim
  Constant11 : Constant  Value=afe_ctrl.i_grid_pos_eta_red_lim
  Constant2 : Constant  Value=afe_ctrl.i_grid_neg_eta_lim
  Constant3 : Constant  Value=afe_ctrl.i_grid_pos_eta_lim
  Constant4 : Constant  Value=0
  Constant5 : Constant  Value=afe_ctrl.i_grid_neg_xi_red_lim
  Constant6 : Constant  Value=0
  Constant7 : Constant  Value=afe_ctrl.i_grid_neg_xi_lim
  Constant8 : Constant  Value=0
  Constant9 : Constant
  Gain : Gain  Gain=frt_data.k_frt_ref
  Gain1 : Gain  Gain=-1
  Gain2 : Gain  Gain=-frt_data.k_frt_ref
  Gain3 : Gain  Gain=frt_data.k_frt_ref
  Gain4 : Gain  Gain=-1
  Gain6 : Gain  Gain=-1
  Saturation Dynamic : sl_discontinuities/Saturation Dynamic  OutMin=[]  OutMax=[]  OutDataTypeStr=Inherit: Same as second input  OutDataType=fixdt(1, 16)  OutScaling=2^-10  DoSatur=off
  Saturation Dynamic1 : sl_discontinuities/Saturation Dynamic  OutMin=[]  OutMax=[]  OutDataTypeStr=Inherit: Same as second input  OutDataType=fixdt(1, 16)  OutScaling=2^-10  DoSatur=off
  Saturation Dynamic2 : sl_discontinuities/Saturation Dynamic  OutMin=[]  OutMax=[]  OutDataTypeStr=Inherit: Same as second input  OutDataType=fixdt(1, 16)  OutScaling=2^-10  DoSatur=off
  Sum{,1..3} (4 alike) : Sum  Inputs=|+-
  Sum4 : Sum  Inputs=++|
  Sum5 : Sum  Inputs=++|
  Sum6 : Sum  Inputs=+-|
  Switch{1..6} (6 alike) : Switch  Threshold=0.5  SaturateOnIntegerOverflow=off  InputSameDT=off
  Terminator : Terminator
  avg_flt_500ms : Subsystem
  avg_flt_500ms1 : Subsystem
  avg_flt_500ms2 : Subsystem
  avg_flt_500ms3 : Subsystem
  positive_reactive_current_reference : Subsystem
  u_161Hz_flt1 : Subsystem
  u_161Hz_flt2 : Subsystem
  u_161Hz_flt3 : Subsystem
  tag scope: i_grid_seq_ref=scoped
  wires:
  positive_reactive_current_reference/1(i_react_pos_ref) -> [i_react_pos_ref]
  Constant9/1 -> Sum6/1
  [frt_active] -> Sum6/2
  u_161Hz_flt1/1(output) -> Bus Creator/1  "i_grid_pos_eta_ref"
  u_161Hz_flt3/1(output) -> Bus Creator/3  "i_grid_neg_xi_ref"
  u_161Hz_flt2/1(output) -> Bus Creator/2  "i_grid_neg_eta_ref"
  Gain6/1 -> Saturation Dynamic2/3
  [red_dyn_active] -> Switch6/2
  Constant5/1 -> Switch6/1
  Switch6/1 -> [i_grid_neg_xi_lim]
  Constant7/1 -> Switch6/3
  Constant4/1 -> [i_react_neg_ref]
  Switch5/1 -> [i_grid_neg_eta_lim]
  Constant1/1 -> Switch5/1
  Constant2/1 -> Switch5/3
  [red_dyn_active] -> Switch5/2
  Saturation Dynamic1/1 -> u_161Hz_flt2/1(input)
  Switch1/1 -> Saturation Dynamic1/2
  [i_grid_neg_eta_lim] -> Saturation Dynamic1/1
  [i_grid_neg_eta_lim] -> Gain4/1
  Gain4/1 -> Saturation Dynamic1/3
  [i_grid_neg_xi_lim] -> Gain6/1
  [i_grid_neg_xi_lim] -> Saturation Dynamic2/1
  Switch3/1 -> Saturation Dynamic2/2
  Saturation Dynamic2/1 -> u_161Hz_flt3/1(input)
  Gain1/1 -> Saturation Dynamic/3
  [i_grid_pos_eta_lim] -> Gain1/1
  [i_grid_pos_eta_lim] -> Saturation Dynamic/1
  Constant11/1 -> Switch4/1
  Constant3/1 -> Switch4/3
  [red_dyn_active] -> Switch4/2
  Switch4/1 -> [i_grid_pos_eta_lim]
  [i_react_neg_ref] -> Sum5/1, Switch1/1
  Sum5/1 -> Switch1/3
  Gain2/1 -> Sum5/2  "di_neg_eta_ref"
  Sum3/1 -> Gain3/1
  Sum6/1 -> Switch3/2, Switch2/2, Switch1/2
  Gain3/1 -> Switch3/3  "di_neg_xi_ref"
  Constant6/1 -> Switch3/1
  Saturation Dynamic/1 -> u_161Hz_flt1/1(input)
  Switch2/1 -> Saturation Dynamic/2
  Sum4/1 -> Switch2/3
  [i_react_pos_ref] -> Sum4/1, Switch2/1
  Gain/1 -> Sum4/2  "dib_pos_eta"
  Bus Creator/1 -> [i_grid_seq_ref]
  In4/1 -> Sum3/1, avg_flt_500ms3/1(In1)  "v_neg_eta"
  avg_flt_500ms2/1(Out1) -> Sum2/2
  In3/1 -> Sum2/1, avg_flt_500ms2/1(In1)  "v_neg_xi"
  Sum2/1 -> Gain2/1
  avg_flt_500ms3/1(Out1) -> Sum3/2
  In2/1 -> Sum1/1, avg_flt_500ms1/1(In1)  "v_pos_eta"
  avg_flt_500ms1/1(Out1) -> Sum1/2
  Sum1/1 -> Terminator/1
  Sum/1 -> Gain/1  "deltaU"
  avg_flt_500ms/1(Out1) -> Sum/2
  In1/1 -> Sum/1, avg_flt_500ms/1(In1)  "v_pos_xi"
  Constant8/1 -> [red_dyn_active]

== system grid_afe_n/afe_abc_mod3/AFE_control/afe_control/current_ctrl/current_transformation ==
  is_a_pu : Inport
  is_b_pu : Inport  Port=2
  is_c_pu : Inport  Port=3
  alphabeta2xieta : MATLAB Function  TreatAsAtomicUnit=on
  uvw2alphabeta : MATLAB Function  TreatAsAtomicUnit=on
  tag scope: id_eta_pu=scoped, id_xi_pu=scoped
  wires:
  is_c_pu/1 -> uvw2alphabeta/3(w)
  alphabeta2xieta/2(eta) -> [id_eta_pu]  "ieta_pu"
  alphabeta2xieta/1(xi) -> [id_xi_pu]  "ixi_pu"
  is_b_pu/1 -> uvw2alphabeta/2(v)
  uvw2alphabeta/2(beta) -> alphabeta2xieta/2(beta)  "ibeta_pu"
  uvw2alphabeta/1(alpha) -> alphabeta2xieta/1(alpha)  "ialpha_pu"
  [phase_grid_pll] -> alphabeta2xieta/3(gamma)
  is_a_pu/1 -> uvw2alphabeta/1(u)

== system grid_afe_n/afe_abc_mod3/AFE_control/afe_control/current_ctrl/inner_current_ctrl ==
  In1 : Inport
  is_abc : Inport  Port=2
  Mux : Mux  Inputs=3
  Selector : Selector  InputPortWidth=3  IndexOptions=Index vector (dialog)  Indices=[1]  OutputSizes=1
  Selector1 : Selector  InputPortWidth=3  IndexOptions=Index vector (dialog)  Indices=[1]  OutputSizes=1
  Selector2 : Selector  InputPortWidth=3  IndexOptions=Index vector (dialog)  Indices=[2]  OutputSizes=1
  Selector3 : Selector  InputPortWidth=3  IndexOptions=Index vector (dialog)  Indices=[2]  OutputSizes=1
  Selector4 : Selector  InputPortWidth=3  IndexOptions=Index vector (dialog)  Indices=[3]  OutputSizes=1
  Selector5 : Selector  InputPortWidth=3  IndexOptions=Index vector (dialog)  Indices=[3]  OutputSizes=1
  isa_ref/isa : Scope  NumInputPorts=2
      settings: ActiveDisplayYMinimum=-3.12274169921875  ActiveDisplayYMaximum=3.67108154296875
  isb_ref/isb : Scope  NumInputPorts=2
      settings: ActiveDisplayYMinimum=-5.0885009765625  ActiveDisplayYMaximum=2.7154541015625  DataLoggingVariableName=ScopeData2
  isc_ref/isc : Scope  NumInputPorts=2
      settings: ActiveDisplayYMinimum=-2.90966796875  ActiveDisplayYMaximum=2.88134765625  DataLoggingVariableName=ScopeData3
  rpi_phase_a : Subsystem
  rpi_phase_b : Subsystem
  rpi_phase_c : Subsystem
  zero_current_ctrl : Subsystem
  uabg : Outport  VectorParamsAs1DForOutWhenUnconnected=off
  tag scope: isa=scoped, isa_ref=scoped, isb=scoped, isb_ref=scoped, isc=scoped, isc_ref=scoped
  wires:
  In1/1 -> Selector4/1, Selector2/1, Selector/1  "id_abc_ref"
  is_abc/1 -> Selector5/1, Selector3/1, Selector1/1  "id_abc"
  Selector/1 -> [isa_ref], isa_ref/isa/1, rpi_phase_a/1(In1)  "isa_ref"
  Selector1/1 -> [isa], isa_ref/isa/2, rpi_phase_a/2(In2)  "isa"
  Selector2/1 -> rpi_phase_b/1(In1), [isb_ref], isb_ref/isb/1  "isb_ref"
  Selector3/1 -> rpi_phase_b/2(In2), [isb], isb_ref/isb/2  "isb"
  Selector4/1 -> rpi_phase_c/1(In1), [isc_ref], isc_ref/isc/1  "isc_ref"
  Selector5/1 -> rpi_phase_c/2(In2), [isc], isc_ref/isc/2  "isc"
  rpi_phase_a/1(Out1) -> Mux/1  "da"
  rpi_phase_b/1(Out1) -> Mux/2  "db"
  rpi_phase_c/1(Out1) -> Mux/3  "dc"
  Mux/1 -> zero_current_ctrl/1(d_abc)  "d_abc"
  zero_current_ctrl/1(u_ctrl_out) -> uabg/1

== system grid_afe_n/afe_abc_mod3/AFE_control/afe_control/current_ctrl/xieta2abc ==
  pos_xi : Inport
  pos_eta : Inport  Port=2
  neg_xi : Inport  Port=3
  neg_eta : Inport  Port=4
  phase : Inport  Port=5
  MATLAB Function2 : MATLAB Function  TreatAsAtomicUnit=on
  Mux : Mux  Inputs=3
  Negative Sequence : MATLAB Function  TreatAsAtomicUnit=on
  Positive Sequence : MATLAB Function  TreatAsAtomicUnit=on
  Sum : Sum  Inputs=|++
  Sum1 : Sum  Inputs=|++
  i_abc : Outport
  wires:
  neg_eta/1 -> Negative Sequence/2(eta)
  MATLAB Function2/1(a) -> Mux/1  "i_a"
  Positive Sequence/2(beta) -> Sum1/1
  Sum/1 -> MATLAB Function2/1(alpha)
  phase/1 -> Negative Sequence/3(phase), Positive Sequence/3(phase)
  MATLAB Function2/3(c) -> Mux/3  "i_c"
  Negative Sequence/1(alpha) -> Sum/2
  Positive Sequence/1(alpha) -> Sum/1
  Negative Sequence/2(beta) -> Sum1/2
  MATLAB Function2/2(b) -> Mux/2  "i_b"
  Sum1/1 -> MATLAB Function2/2(beta)
  neg_xi/1 -> Negative Sequence/1(xi)
  pos_xi/1 -> Positive Sequence/1(xi)
  pos_eta/1 -> Positive Sequence/2(eta)
  Mux/1 -> i_abc/1  "i_abc"

== system grid_afe_n/afe_abc_mod3/AFE_control/afe_control/data_to_worspace_module_1/dq_pll ==
  Bus Creator1 : BusCreator  Inputs=8
  dqPLLs : Outport
  wires:
  [phase_grid_fht_simulink_pll] -> Bus Creator1/5  "phase_grid_fht_simulink_pll"
  [omega_grid_fht_simulink_pll] -> Bus Creator1/6  "omega_grid_fht_simulink_pll"
  [omega_grid_fhtsr_dqpll] -> Bus Creator1/8  "omega_grid_fhtsr_dqpll"
  [phase_grid_fhtsr_dqpll] -> Bus Creator1/7  "phase_grid_fhtsr_dqpll"
  [omega_grid_dqpll_ccaller] -> Bus Creator1/4  "omega_grid_dqpll_ccaller"
  [phase_grid_dqpll_ccaller] -> Bus Creator1/3  "phase_grid_dqpll_ccaller"
  [omega_grid_pu_dqpll] -> Bus Creator1/2  "omega_grid_pu_dqpll"
  [phase_grid_dqpll] -> Bus Creator1/1  "phase_grid_dqpll"
  Bus Creator1/1 -> dqPLLs/1

== system grid_afe_n/afe_abc_mod3/AFE_control/afe_control/data_to_worspace_module_1/inner_current_tracking ==
  Bus Creator1 : BusCreator  Inputs=11
  m_inner_current_tracking : Outport
  wires:
  [iz_pu] -> Bus Creator1/10  "iz_pu"
  [id_eta_pu] -> Bus Creator1/2  "i_eta_pu"
  [isc] -> Bus Creator1/8  "isc_pu"
  [isa_ref] -> Bus Creator1/3  "isa_pu_ref"
  [isa] -> Bus Creator1/4  "isa_pu"
  [id_xi_pu] -> Bus Creator1/1  "i_xi_pu"
  [iz_pu_ref] -> Bus Creator1/9  "iz_pu_ref"
  [isb] -> Bus Creator1/6  "isb_pu"
  [isb_ref] -> Bus Creator1/5  "isb_pu_ref"
  [iz_ctrl_out] -> Bus Creator1/11  "iz_ctrl_out"
  [isc_ref] -> Bus Creator1/7  "isc_pu_ref"
  Bus Creator1/1 -> m_inner_current_tracking/1

== system grid_afe_n/afe_abc_mod3/AFE_control/afe_control/data_to_worspace_module_1/pwr_meter ==
  Bus Creator1 : BusCreator  Inputs=4
  m_pwr_meter : Outport
  wires:
  [u_grid_pu_rms] -> Bus Creator1/2  "u_grid_pu_rms"
  Bus Creator1/1 -> m_pwr_meter/1
  [pwr_act_grid] -> Bus Creator1/3  "pwr_act_grid"
  [pwr_react_grid] -> Bus Creator1/4  "pwr_react_grid"
  [i_grid_pu_rms] -> Bus Creator1/1  "i_grid_pu_rms"

== system grid_afe_n/afe_abc_mod3/AFE_control/afe_control/data_to_worspace_module_1/sequences_data ==
  Bus Creator1 : BusCreator  Inputs=11
  Bus Selector : BusSelector  OutputSignals=i_grid_pos_eta_ref,i_grid_neg_eta_ref,i_grid_neg_xi_ref
  m_seq : Outport
  wires:
  [i_grid_neg_eta_avg] -> Bus Creator1/11  "i_grid_neg_eta_avg"
  [i_grid_neg_xi_avg] -> Bus Creator1/10  "i_grid_neg_xi_avg"
  [i_grid_pos_eta_avg] -> Bus Creator1/9  "i_grid_pos_eta_avg"
  [i_grid_pos_xi_avg] -> Bus Creator1/8  "i_grid_pos_xi_avg"
  [v_grid_neg_eta_avg] -> Bus Creator1/7  "v_grid_neg_eta_avg"
  [v_grid_neg_xi_avg] -> Bus Creator1/6  "v_grid_neg_xi_avg"
  [v_grid_pos_eta_avg] -> Bus Creator1/5  "v_grid_pos_eta_avg"
  [v_grid_pos_xi_avg] -> Bus Creator1/4  "v_grid_pos_xi_avg"
  Bus Selector/1 -> Bus Creator1/1  "<i_grid_pos_eta_ref>"
  Bus Selector/2 -> Bus Creator1/2  "<i_grid_neg_eta_ref>"
  Bus Selector/3 -> Bus Creator1/3  "<i_grid_neg_xi_ref>"
  [i_grid_seq_ref] -> Bus Selector/1
  Bus Creator1/1 -> m_seq/1
